simulink model "stereo_camera_q_dot"  (R2025b)
settings: Solver=FixedStepDiscrete  StartTime=0  StopTime=inf  FixedStep=Ts  RelTol=1e-3
InitFcn:
  | % 获取当前.slx模型所在文件夹
  | model_path = fileparts(which(gcs));
  | % 向上跳转、拼接目标函数所在文件夹（根据你的目录调整）
  | func_folder = fullfile(model_path,'..', 'config');
  | % 添加到搜索路径
  | addpath(func_folder);
  | % 执行初始化函数
  | init_single_camera_q_dot_tracking;
undefined symbols (not defined in the file or in its folder): camera_velocity_feedback_timeout_sec, controller_enable, cx, cy, data, data_SL_Info, depth_safe_max, depth_safe_min, depth_safety_gain, ekf_gate_threshold, enable_ekf_feedforward, enable_proportional, fx, fy, joint_acceleration_limit, joint_nominal_configuration, joint_position_max, joint_position_min, joint_soft_margin, joint_state_timeout_sec, joint_velocity_limit, k_ff, Kpx, Kpy, measurement_reset_timeout, nullspace_posture_gain, P0, Publish, Q_ekf, R_ekf, required_valid_frames, ros, ros2lib, singularity_sigma_stop, singularity_sigma_warn, Subscribe, target_timeout_sec, task_velocity_filter_tau, Ts, visual_damping_max, visual_damping_min, visual_min_depth, Z_hat
libraries: robotmaniplib x2
(part 1 of 2)
Description:
  | Fixed-focus monocular XY target tracking. Outputs camera-frame [vx vy 0 0 0 0]; robot kinematics remain external.
settings Model: DataDictionary=ros2lib.sldd  Creator=ASUS  LastModifiedBy=harry
settings DataIOCC: SignalLogging=off

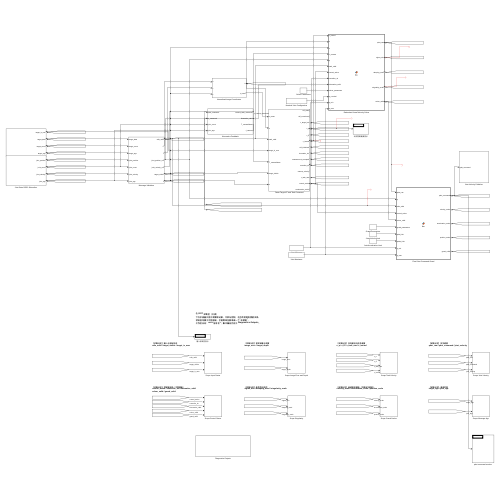
[thumbnail: Simulink's stored preview of the top-level diagram]
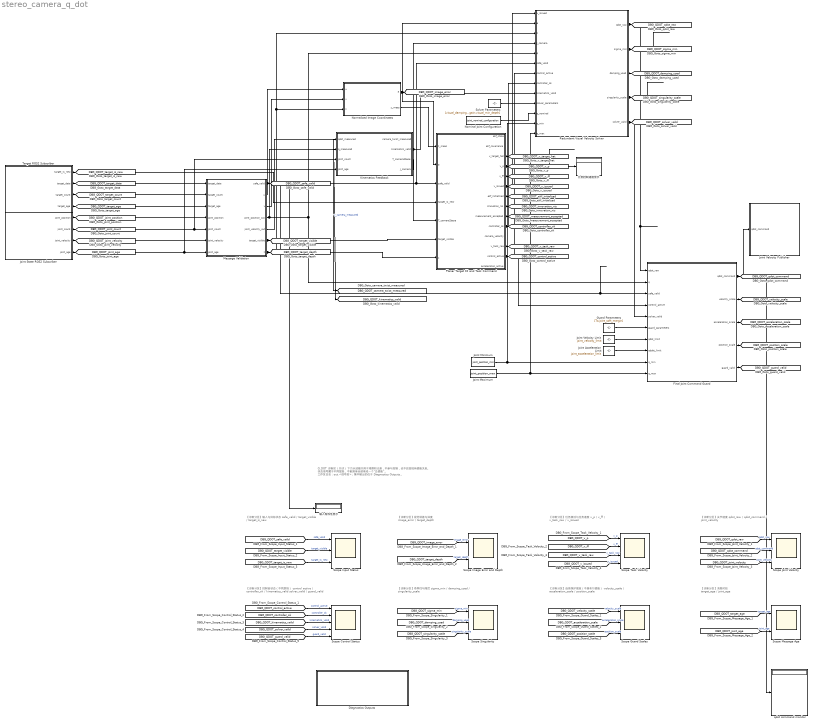
== system stereo_camera_q_dot ==
  note: Q_DOT 诊断区（只读）
      | 下方示波器只用于观察和记录，不参与控制，也不改变现有使能关系。
      | 状态信号属于不同层级，不能简单全部串成一个“总使能”。
      | 工作区日志：out.<信号名>；集中输出仍位于 Diagnostics Outputs。
  note: 【诊断分区】输入与目标状态
      | safe_valid / target_visible / target_is_new
  note: 【诊断分区】视觉误差与深度
      | image_error / target_depth
  note: 【诊断分区】任务激活与任务速度
      | v_p / v_ff / v_task_raw / v_issued
  note: 【诊断分区】关节速度
      | qdot_raw / qdot_command / joint_velocity
  note: 【诊断分区】控制链状态（不同层级）
      | control_active / controller_ok / kinematics_valid
      | solver_valid / guard_valid
  note: 【诊断分区】奇异性与阻尼
      | sigma_min / damping_used / singularity_scale
  note: 【诊断分区】连续保护缩放（不是布尔使能）
      | velocity_scale / acceleration_scale / position_scale
  note: 【诊断分区】消息时效
      | target_age / joint_age
  Diagnostics Outputs : Subsystem
  Final Joint Command Guard : MATLAB Function  TreatAsAtomicUnit=on
  Guard Parameters : Constant  Value=[Ts;joint_soft_margin]
  Joint Acceleration Limit : Constant  Value=joint_acceleration_limit
  Joint Maximum : Constant  Value=joint_position_max
  Joint Minimum : Constant  Value=joint_position_min
  Joint State ROS2 Subscriber : Subsystem
  Joint Velocity Limit : Constant  Value=joint_velocity_limit
  Joint Velocity Publisher : Subsystem
  Kinematics Feedback : Subsystem
  Message Validation : Subsystem
  Nominal Joint Configuration : Constant  Value=joint_nominal_configuration
  Normalized Image Coordinates : Subsystem
  Planar Target KF and Task Command : Subsystem
  Redundant Visual Velocity Solver : MATLAB Function  TreatAsAtomicUnit=on
  Scope Control Status : Scope  NumInputPorts=5
      settings: TimeSpan=10  ActiveDisplayString=5  Title=guard_valid  ActiveDisplayYMinimum=-0.037001953201183713  ActiveDisplayYMaximum=0.0101088347899616  DataLoggingVariableName=ScopeData4
  Scope Guard Scales : Scope  NumInputPorts=3
      settings: TimeSpan=10  ActiveDisplayString=3  Title=position_scale  ActiveDisplayYMinimum=-12.068513318672558  ActiveDisplayYMaximum=6.6876450330275015  DataLoggingVariableName=ScopeData6
  Scope Image Error and Depth : Scope  NumInputPorts=2
      settings: TimeSpan=10  Title=target_depth  ActiveDisplayYMinimum=-1  ActiveDisplayYMaximum=1
  Scope Input Status : Scope  NumInputPorts=3
      settings: TimeSpan=10  ActiveDisplayString=3  Title=target_is_new  ActiveDisplayYMinimum=-1.6084422447956979  ActiveDisplayYMaximum=1.406793571934575  DataLoggingVariableName=ScopeData7
  Scope Joint Velocity : Scope  NumInputPorts=3
      settings: TimeSpan=10  ActiveDisplayString=3  Title=joint_velocity  ActiveDisplayYMinimum=-1.0517167509781138  ActiveDisplayYMaximum=1.0307773782957734  DataLoggingVariableName=ScopeData2
  Scope Message Age : Scope  NumInputPorts=2
      settings: TimeSpan=10  Title=joint_age  ActiveDisplayYMinimum=-1  ActiveDisplayYMaximum=1
  Scope Singularity : Scope  NumInputPorts=3
      settings: TimeSpan=10  ActiveDisplayString=3  Title=singularity_scale  ActiveDisplayYMinimum=-3.3735923675324466  ActiveDisplayYMaximum=2.902388236211491  DataLoggingVariableName=ScopeData5
  Scope Task Velocity : Scope  NumInputPorts=4
      settings: TimeSpan=10  ActiveDisplayString=4  Title=v_issued  ActiveDisplayYMinimum=-1  ActiveDisplayYMaximum=1  DataLoggingVariableName=ScopeData3
  Solver Parameters : Constant  Value=[visual_damping_min;visual_damping_max;singularity_sigma_stop;singularity_sigma_warn;nullspace_posture_gain;depth_safe_min;depth_safe_max;depth_safety_gain;visual_min_depth]
  Target ROS2 Subscriber : Subsystem
  qdot command monitor : Display
  比例控制速度显示 : Display
  输入有效性显示 : Display
  tag scope: DBG_QDOT_acceleration_scale=global, DBG_QDOT_camera_twist_measured=global, DBG_QDOT_control_active=global, DBG_QDOT_controller_ok=global, DBG_QDOT_damping_used=global, DBG_QDOT_ekf_initialized=global, DBG_QDOT_guard_valid=global, DBG_QDOT_image_error=global, DBG_QDOT_innovation_nis=global, DBG_QDOT_joint_age=global, DBG_QDOT_joint_count=global, DBG_QDOT_joint_position=global, DBG_QDOT_joint_velocity=global, DBG_QDOT_kinematics_valid=global, DBG_QDOT_measurement_accepted=global, DBG_QDOT_position_scale=global, DBG_QDOT_qdot_command=global, DBG_QDOT_qdot_raw=global, DBG_QDOT_safe_valid=global, DBG_QDOT_sigma_min=global, DBG_QDOT_singularity_scale=global, DBG_QDOT_solver_valid=global, DBG_QDOT_target_age=global, DBG_QDOT_target_count=global, DBG_QDOT_target_data=global, DBG_QDOT_target_depth=global, DBG_QDOT_target_is_new=global, DBG_QDOT_target_visible=global, DBG_QDOT_v_ff=global, DBG_QDOT_v_issued=global, DBG_QDOT_v_p=global, DBG_QDOT_v_target_hat=global, DBG_QDOT_v_task_raw=global, DBG_QDOT_velocity_scale=global
  wires:
  Final Joint Command Guard/1(qdot_command) -> Joint Velocity Publisher/1(qdot_command), qdot command monitor/1, [DBG_QDOT_qdot_command]
  Message Validation/4(joint_position_out) -> Final Joint Command Guard/2(q), Redundant Visual Velocity Solver/5(q), Kinematics Feedback/2(q_measured)
  Kinematics Feedback/2(kinematics_valid) -> Redundant Visual Velocity Solver/9(kinematics_valid), [DBG_QDOT_kinematics_valid]
  Joint Velocity Limit/1 -> Final Joint Command Guard/7(qdot_limit)
  Message Validation/2(u) -> Normalized Image Coordinates/1(u)
  Target ROS2 Subscriber/3(target_count) -> Message Validation/2(target_count), [DBG_QDOT_target_count]
  Redundant Visual Velocity Solver/5(solver_valid) -> Final Joint Command Guard/5(solver_valid), [DBG_QDOT_solver_valid]
  Target ROS2 Subscriber/1(target_is_new) -> Planar Target KF and Task Command/4(target_is_new), [DBG_QDOT_target_is_new]
  Planar Target KF and Task Command/10(controller_ok) -> Redundant Visual Velocity Solver/8(controller_ok), [DBG_QDOT_controller_ok]
  Message Validation/5(joint_velocity_out) -> Kinematics Feedback/1(qdot_measured)
  Message Validation/7(z) -> Redundant Visual Velocity Solver/3(z), Normalized Image Coordinates/3(z), Planar Target KF and Task Command/7(z), [DBG_QDOT_target_depth]
  Joint Acceleration Limit/1 -> Final Joint Command Guard/8(qddot_limit)
  Joint State ROS2 Subscriber/4(joint_age) -> Kinematics Feedback/4(joint_age), Message Validation/7(joint_age), [DBG_QDOT_joint_age]
  Joint State ROS2 Subscriber/3(joint_velocity) -> Message Validation/6(joint_velocity), [DBG_QDOT_joint_velocity]
  Message Validation/6(target_visible) -> Planar Target KF and Task Command/6(target_visible), [DBG_QDOT_target_visible]
  Kinematics Feedback/4(J_camera) -> Redundant Visual Velocity Solver/4(J_camera)
  Redundant Visual Velocity Solver/1(qdot_raw) -> [DBG_QDOT_qdot_raw], Final Joint Command Guard/1(qdot_raw)
  Message Validation/1(safe_valid) -> Final Joint Command Guard/3(safe_valid), Redundant Visual Velocity Solver/6(safe_valid), Planar Target KF and Task Command/3(safe_valid), 输入有效性显示/1, [DBG_QDOT_safe_valid]
  Message Validation/3(v) -> Normalized Image Coordinates/2(v)
  Planar Target KF and Task Command/13(control_active) -> Redundant Visual Velocity Solver/7(control_active), Final Joint Command Guard/4(control_active), [DBG_QDOT_control_active]
  Joint State ROS2 Subscriber/1(joint_position) -> Message Validation/4(joint_position), [DBG_QDOT_joint_position]
  Guard Parameters/1 -> Final Joint Command Guard/6(guard_parameters)
  Joint State ROS2 Subscriber/2(joint_count) -> Kinematics Feedback/3(joint_count), Message Validation/5(joint_count), [DBG_QDOT_joint_count]
  Normalized Image Coordinates/1(e) -> Planar Target KF and Task Command/2(e), Redundant Visual Velocity Solver/2(e), [DBG_QDOT_image_error]
  Target ROS2 Subscriber/2(target_data) -> Message Validation/1(target_data), [DBG_QDOT_target_data]
  Normalized Image Coordinates/2(z_meas) -> Planar Target KF and Task Command/1(z_meas)
  Kinematics Feedback/3(T_camera2base) -> Planar Target KF and Task Command/5(T_camera2base)
  Solver Parameters/1 -> Redundant Visual Velocity Solver/10(solver_parameters)
  Nominal Joint Configuration/1 -> Redundant Visual Velocity Solver/11(q_nominal)
  Joint Minimum/1 -> Redundant Visual Velocity Solver/12(q_min), Final Joint Command Guard/9(q_min)
  Joint Maximum/1 -> Final Joint Command Guard/10(q_max), Redundant Visual Velocity Solver/13(q_max)
  Target ROS2 Subscriber/4(target_age) -> Message Validation/3(target_age), [DBG_QDOT_target_age]
  Planar Target KF and Task Command/4(v_p) -> 比例控制速度显示/1, [DBG_QDOT_v_p]
  Planar Target KF and Task Command/6(v_issued) -> Redundant Visual Velocity Solver/1(v_issued), [DBG_QDOT_v_issued]
  Redundant Visual Velocity Solver/2(sigma_min) -> [DBG_QDOT_sigma_min]
  Redundant Visual Velocity Solver/4(singularity_scale) -> [DBG_QDOT_singularity_scale]
  Kinematics Feedback/1(camera_twist_measured) -> [DBG_QDOT_camera_twist_measured]  "v_camera_measured"
  Planar Target KF and Task Command/3(v_target_hat) -> [DBG_QDOT_v_target_hat]
  Planar Target KF and Task Command/5(v_ff) -> [DBG_QDOT_v_ff]
  Planar Target KF and Task Command/7(ekf_initialized) -> [DBG_QDOT_ekf_initialized]
  Planar Target KF and Task Command/8(innovation_nis) -> [DBG_QDOT_innovation_nis]
  Planar Target KF and Task Command/9(measurement_accepted) -> [DBG_QDOT_measurement_accepted]
  Planar Target KF and Task Command/12(v_task_raw) -> [DBG_QDOT_v_task_raw]
  Redundant Visual Velocity Solver/3(damping_used) -> [DBG_QDOT_damping_used]
  Final Joint Command Guard/2(velocity_scale) -> [DBG_QDOT_velocity_scale]
  Final Joint Command Guard/3(acceleration_scale) -> [DBG_QDOT_acceleration_scale]
  Final Joint Command Guard/4(position_scale) -> [DBG_QDOT_position_scale]
  Final Joint Command Guard/5(guard_valid) -> [DBG_QDOT_guard_valid]
  [DBG_QDOT_safe_valid] -> Scope Input Status/1  "safe_valid"
  [DBG_QDOT_target_visible] -> Scope Input Status/2  "target_visible"
  [DBG_QDOT_target_is_new] -> Scope Input Status/3  "target_is_new"
  [DBG_QDOT_image_error] -> Scope Image Error and Depth/1  "image_error"
  [DBG_QDOT_target_depth] -> Scope Image Error and Depth/2  "target_depth"
  [DBG_QDOT_v_p] -> Scope Task Velocity/1  "v_p"
  [DBG_QDOT_v_ff] -> Scope Task Velocity/2  "v_ff"
  [DBG_QDOT_v_task_raw] -> Scope Task Velocity/3  "v_task_raw"
  [DBG_QDOT_v_issued] -> Scope Task Velocity/4  "v_issued"
  [DBG_QDOT_qdot_raw] -> Scope Joint Velocity/1  "qdot_raw"
  [DBG_QDOT_qdot_command] -> Scope Joint Velocity/2  "qdot_command"
  [DBG_QDOT_joint_velocity] -> Scope Joint Velocity/3  "joint_velocity"
  [DBG_QDOT_control_active] -> Scope Control Status/1  "control_active"
  [DBG_QDOT_controller_ok] -> Scope Control Status/2  "controller_ok"
  [DBG_QDOT_kinematics_valid] -> Scope Control Status/3  "kinematics_valid"
  [DBG_QDOT_solver_valid] -> Scope Control Status/4  "solver_valid"
  [DBG_QDOT_guard_valid] -> Scope Control Status/5  "guard_valid"
  [DBG_QDOT_sigma_min] -> Scope Singularity/1  "sigma_min"
  [DBG_QDOT_damping_used] -> Scope Singularity/2  "damping_used"
  [DBG_QDOT_singularity_scale] -> Scope Singularity/3  "singularity_scale"
  [DBG_QDOT_velocity_scale] -> Scope Guard Scales/1  "velocity_scale"
  [DBG_QDOT_acceleration_scale] -> Scope Guard Scales/2  "acceleration_scale"
  [DBG_QDOT_position_scale] -> Scope Guard Scales/3  "position_scale"
  [DBG_QDOT_target_age] -> Scope Message Age/1  "target_age"
  [DBG_QDOT_joint_age] -> Scope Message Age/2  "joint_age"

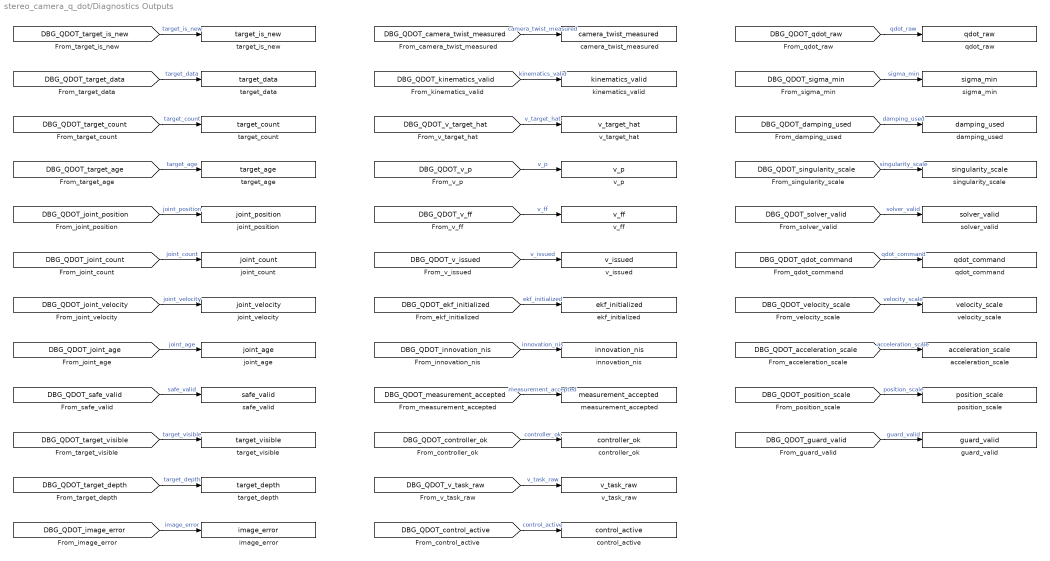
== system stereo_camera_q_dot/Diagnostics Outputs ==
  acceleration_scale : ToWorkspace  VariableName=acceleration_scale  SaveFormat=Timeseries  SampleTime=-1
  camera_twist_measured : ToWorkspace  VariableName=camera_twist_measured  SaveFormat=Timeseries  SampleTime=-1
  control_active : ToWorkspace  VariableName=control_active  SaveFormat=Timeseries  SampleTime=-1
  controller_ok : ToWorkspace  VariableName=controller_ok  SaveFormat=Timeseries  SampleTime=-1
  damping_used : ToWorkspace  VariableName=damping_used  SaveFormat=Timeseries  SampleTime=-1
  ekf_initialized : ToWorkspace  VariableName=ekf_initialized  SaveFormat=Timeseries  SampleTime=-1
  guard_valid : ToWorkspace  VariableName=guard_valid  SaveFormat=Timeseries  SampleTime=-1
  image_error : ToWorkspace  VariableName=image_error  SaveFormat=Timeseries  SampleTime=-1
  innovation_nis : ToWorkspace  VariableName=innovation_nis  SaveFormat=Timeseries  SampleTime=-1
  joint_age : ToWorkspace  VariableName=joint_age  SaveFormat=Timeseries  SampleTime=-1
  joint_count : ToWorkspace  VariableName=joint_count  SaveFormat=Timeseries  SampleTime=-1
  joint_position : ToWorkspace  VariableName=joint_position  SaveFormat=Timeseries  SampleTime=-1
  joint_velocity : ToWorkspace  VariableName=joint_velocity  SaveFormat=Timeseries  SampleTime=-1
  kinematics_valid : ToWorkspace  VariableName=kinematics_valid  SaveFormat=Timeseries  SampleTime=-1
  measurement_accepted : ToWorkspace  VariableName=measurement_accepted  SaveFormat=Timeseries  SampleTime=-1
  position_scale : ToWorkspace  VariableName=position_scale  SaveFormat=Timeseries  SampleTime=-1
  qdot_command : ToWorkspace  VariableName=qdot_command  SaveFormat=Timeseries  SampleTime=-1
  qdot_raw : ToWorkspace  VariableName=qdot_raw  SaveFormat=Timeseries  SampleTime=-1
  safe_valid : ToWorkspace  VariableName=safe_valid  SaveFormat=Timeseries  SampleTime=-1
  sigma_min : ToWorkspace  VariableName=sigma_min  SaveFormat=Timeseries  SampleTime=-1
  singularity_scale : ToWorkspace  VariableName=singularity_scale  SaveFormat=Timeseries  SampleTime=-1
  solver_valid : ToWorkspace  VariableName=solver_valid  SaveFormat=Timeseries  SampleTime=-1
  target_age : ToWorkspace  VariableName=target_age  SaveFormat=Timeseries  SampleTime=-1
  target_count : ToWorkspace  VariableName=target_count  SaveFormat=Timeseries  SampleTime=-1
  target_data : ToWorkspace  VariableName=target_data  SaveFormat=Timeseries  SampleTime=-1
  target_depth : ToWorkspace  VariableName=target_depth  SaveFormat=Timeseries  SampleTime=-1
  target_is_new : ToWorkspace  VariableName=target_is_new  SaveFormat=Timeseries  SampleTime=-1
  target_visible : ToWorkspace  VariableName=target_visible  SaveFormat=Timeseries  SampleTime=-1
  v_ff : ToWorkspace  VariableName=v_ff  SaveFormat=Timeseries  SampleTime=-1
  v_issued : ToWorkspace  VariableName=v_issued  SaveFormat=Timeseries  SampleTime=-1
  v_p : ToWorkspace  VariableName=v_p  SaveFormat=Timeseries  SampleTime=-1
  v_target_hat : ToWorkspace  VariableName=v_target_hat  SaveFormat=Timeseries  SampleTime=-1
  v_task_raw : ToWorkspace  VariableName=v_task_raw  SaveFormat=Timeseries  SampleTime=-1
  velocity_scale : ToWorkspace  VariableName=velocity_scale  SaveFormat=Timeseries  SampleTime=-1
  wires:
  [DBG_QDOT_target_is_new] -> target_is_new/1  "target_is_new"
  [DBG_QDOT_target_data] -> target_data/1  "target_data"
  [DBG_QDOT_target_count] -> target_count/1  "target_count"
  [DBG_QDOT_target_age] -> target_age/1  "target_age"
  [DBG_QDOT_joint_position] -> joint_position/1  "joint_position"
  [DBG_QDOT_joint_count] -> joint_count/1  "joint_count"
  [DBG_QDOT_joint_velocity] -> joint_velocity/1  "joint_velocity"
  [DBG_QDOT_joint_age] -> joint_age/1  "joint_age"
  [DBG_QDOT_safe_valid] -> safe_valid/1  "safe_valid"
  [DBG_QDOT_target_visible] -> target_visible/1  "target_visible"
  [DBG_QDOT_target_depth] -> target_depth/1  "target_depth"
  [DBG_QDOT_image_error] -> image_error/1  "image_error"
  [DBG_QDOT_camera_twist_measured] -> camera_twist_measured/1  "camera_twist_measured"
  [DBG_QDOT_kinematics_valid] -> kinematics_valid/1  "kinematics_valid"
  [DBG_QDOT_v_target_hat] -> v_target_hat/1  "v_target_hat"
  [DBG_QDOT_v_p] -> v_p/1  "v_p"
  [DBG_QDOT_v_ff] -> v_ff/1  "v_ff"
  [DBG_QDOT_v_issued] -> v_issued/1  "v_issued"
  [DBG_QDOT_ekf_initialized] -> ekf_initialized/1  "ekf_initialized"
  [DBG_QDOT_innovation_nis] -> innovation_nis/1  "innovation_nis"
  [DBG_QDOT_measurement_accepted] -> measurement_accepted/1  "measurement_accepted"
  [DBG_QDOT_controller_ok] -> controller_ok/1  "controller_ok"
  [DBG_QDOT_v_task_raw] -> v_task_raw/1  "v_task_raw"
  [DBG_QDOT_control_active] -> control_active/1  "control_active"
  [DBG_QDOT_qdot_raw] -> qdot_raw/1  "qdot_raw"
  [DBG_QDOT_sigma_min] -> sigma_min/1  "sigma_min"
  [DBG_QDOT_damping_used] -> damping_used/1  "damping_used"
  [DBG_QDOT_singularity_scale] -> singularity_scale/1  "singularity_scale"
  [DBG_QDOT_solver_valid] -> solver_valid/1  "solver_valid"
  [DBG_QDOT_qdot_command] -> qdot_command/1  "qdot_command"
  [DBG_QDOT_velocity_scale] -> velocity_scale/1  "velocity_scale"
  [DBG_QDOT_acceleration_scale] -> acceleration_scale/1  "acceleration_scale"
  [DBG_QDOT_position_scale] -> position_scale/1  "position_scale"
  [DBG_QDOT_guard_valid] -> guard_valid/1  "guard_valid"

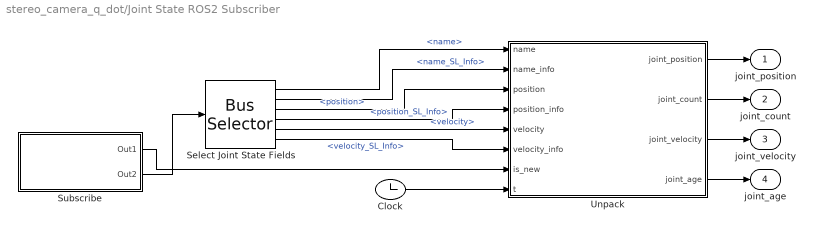
== system stereo_camera_q_dot/Joint State ROS2 Subscriber ==
  Clock : Clock
  Select Joint State Fields : BusSelector  OutputSignals=name,name_SL_Info,position,position_SL_Info,velocity,velocity_SL_Info
  Subscribe : Subsystem  AncestorBlock=ros2lib/Subscribe  LoadFcn=ros.slros2.internal.block.SubscribeBlockMask.messageLoadFcn(gcb);  InitFcn=ros.slros.internal.block.errorIfBlocksConflict(bdroot(gcb));  mask(ROS2 Subscribe){topicSource=Select from ROS network, topic=/franka/joint_states, messageType=sensor_msgs/JointState, sampleTime=Ts, QOSHistory=Keep last, QOSDepth=1, QOSReliability=Best effort, QOSDurability=Volatile, QOSDeadline=Inf, QOSLifespan=Inf, QOSLiveliness=Automatic, QOSLeaseDuration=Inf, QOSAvoidROSNamespaceConventions=off}
      mask prompts: topicSource "ros:slros:blockmask:TopicSourcePrompt"; topic "ros:slros:blockmask:TopicPrompt"; messageType "ros:slros:blockmask:MessageTypePrompt"; sampleTime "ros:slros:blockmask:SampleTimePrompt"; QOSHistory "ros:slros2:blockmask:QOSHistoryPrompt"; QOSDepth "ros:slros2:blockmask:QOSDepthPrompt"; QOSReliability "ros:slros2:blockmask:QOSReliabilityPrompt"; QOSDurability "ros:slros2:blockmask:QOSDurabilityPrompt"; QOSDeadline "ros:slros2:blockmask:QOSDeadlinePrompt"; QOSLifespan "ros:slros2:blockmask:QOSLifespanPrompt"; QOSLiveliness "ros:slros2:blockmask:QOSLivelinessPrompt"; QOSLeaseDuration "ros:slros2:blockmask:QOSLeaseDurationPrompt"; QOSAvoidROSNamespaceConventions "ros:slros2:blockmask:QOSAvoidROSNamespaceConventionsPrompt"
      mask help: ros:slros:blockmask:SubscriberDescription
      mask init:
      | ros.slros2.internal.block.SubscribeBlockMask.dispatch('maskInitialize', gcb);
      settings: ModelCloseFcn=ros.slros2.internal.bus.Util.clearSLBusesInGlobalScope(gcb);
      mask Help: eval('ros.slros.internal.helpview(''ros2SubscribeBlock'')');
      mask TypeOptions topicSource: ros:slros2:blockmask:TopicSourceFromNetwork | ros:slros2:blockmask:TopicSourceSpecifyOwn
      mask Callback topicSource: ros.slros2.internal.block.SubscribeBlockMask.dispatch('topicSourceSelect', gcb);
      mask Callback topic: ros.slros2.internal.block.SubscribeBlockMask.dispatch('topicEdit', gcb);
      mask Callback messageType: ros.slros2.internal.block.SubscribeBlockMask.dispatch('messageTypeEdit', gcb);
      mask TypeOptions sampleTime: Constant/SampleTime
      mask TypeOptions QOSHistory: SourceBlock/QOSHistory
      mask Callback QOSHistory: ros.slros2.internal.block.QOSSettingsMask.qosHistorySelect(gcb);
      mask TypeOptions QOSDepth: SourceBlock/QOSDepth
      mask TypeOptions QOSReliability: SourceBlock/QOSReliability
      mask TypeOptions QOSDurability: SourceBlock/QOSDurability
      mask TypeOptions QOSDeadline: SourceBlock/QOSDeadline
      mask TypeOptions QOSLifespan: SourceBlock/QOSLifespan
      mask TypeOptions QOSLiveliness: SourceBlock/QOSLiveliness
      mask TypeOptions QOSLeaseDuration: SourceBlock/QOSLeaseDuration
      mask TypeOptions QOSAvoidROSNamespaceConventions: SourceBlock/QOSAvoidROSNamespaceConventions
      mask DialogControl id_netAddrLink Prompt: ros:slros2:blockmask:ConfigNetworkAddrLinkText
      mask DialogControl id_netAddrLink Callback: ros.slros2.internal.block.SubscribeBlockMask.dispatch('configureNetworkAddrDlg', gcb);
      mask DialogControl Container13 Prompt: ros:slros2:blockmask:PubSubMainTab
      mask DialogControl topicSource Prompt: Topic source:
      mask DialogControl topic Prompt: Topic:
      mask DialogControl id_topicSelectBtn Prompt: ros:slros:blockmask:SelectPrompt
      mask DialogControl id_topicSelectBtn Callback: ros.slros2.internal.block.SubscribeBlockMask.dispatch('topicSelect', gcb, 'ros.slros2.internal.dlg.TopicSelector');
      mask DialogControl messageType Prompt: Message type:
      mask DialogControl id_msgTypeSelectBtn Prompt: ros:slros:blockmask:SelectPrompt
      mask DialogControl id_msgTypeSelectBtn Callback: ros.slros2.internal.block.SubscribeBlockMask.dispatch('messageTypeSelect', gcb, 'ros.slros2.internal.dlg.MessageTypeSelector');
      mask DialogControl sampleTime Prompt: Sample time:
      mask DialogControl id_cgContainer Prompt: ros:slros2:blockmask:PubSubQOSTab
      mask DialogControl QOSHistory Prompt: History:
      mask DialogControl QOSDepth Prompt: Depth:
      mask DialogControl QOSReliability Prompt: Reliability:
      mask DialogControl QOSDurability Prompt: Durability:
      mask DialogControl QOSDeadline Prompt: Deadline:
      mask DialogControl QOSLifespan Prompt: Lifespan:
      mask DialogControl QOSLiveliness Prompt: Liveliness:
      mask DialogControl QOSLeaseDuration Prompt: Lease Duration:
      mask DialogControl QOSAvoidROSNamespaceConventions Prompt: Avoid ROS Namespace Conventions
      mask Display:
      | color('black');
      | text(0.83, 0.15, '/franka/joint_states', 'horizontalAlignment', 'right');
      | port_label('output', 1, 'IsNew');
      | port_label('output', 2, 'Msg');
  Unpack : MATLAB Function  TreatAsAtomicUnit=on
  joint_position : Outport
  joint_count : Outport  Port=2
  joint_velocity : Outport  Port=3
  joint_age : Outport  Port=4
  wires:
  Unpack/1(joint_position) -> joint_position/1
  Unpack/2(joint_count) -> joint_count/1
  Unpack/3(joint_velocity) -> joint_velocity/1
  Unpack/4(joint_age) -> joint_age/1
  Subscribe/2(Out2) -> Select Joint State Fields/1
  Select Joint State Fields/1 -> Unpack/1(name)  "<name>"
  Select Joint State Fields/2 -> Unpack/2(name_info)  "<name_SL_Info>"
  Select Joint State Fields/3 -> Unpack/3(position)  "<position>"
  Select Joint State Fields/4 -> Unpack/4(position_info)  "<position_SL_Info>"
  Select Joint State Fields/5 -> Unpack/5(velocity)  "<velocity>"
  Select Joint State Fields/6 -> Unpack/6(velocity_info)  "<velocity_SL_Info>"
  Subscribe/1(Out1) -> Unpack/7(is_new)
  Clock/1 -> Unpack/8(t)

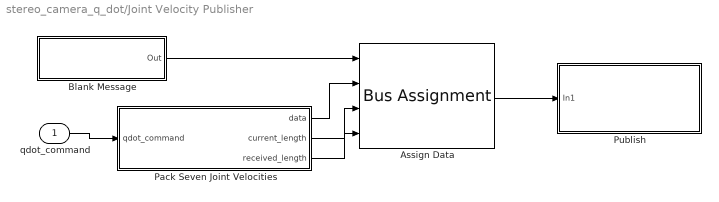
== system stereo_camera_q_dot/Joint Velocity Publisher ==
  qdot_command : Inport
  Assign Data : BusAssignment  AssignedSignals=data,data_SL_Info.CurrentLength,data_SL_Info.ReceivedLength
  Blank Message : Subsystem  AncestorBlock=ros2lib/Blank Message  LoadFcn=ros.slros2.internal.block.MessageBlockMask.messageLoadFcn(gcb);  InitFcn=ros.slros.internal.block.errorIfBlocksConflict(bdroot(gcb));  mask(ROS2 Blank Message){messageClass=Message, entityType=std_msgs/Float64MultiArray, messageType=std_msgs/Float64MultiArray, SampleTime=Ts}
      mask prompts: messageClass "ros:slros:blockmask:MessageClassPrompt"; entityType "ros:slros:blockmask:TypePrompt"; messageType "ros:slros:blockmask:FullTypePrompt"; SampleTime "Simulink:blkprm_prompts:AllSrcBlksSampleTime"
      mask help: ros:slros2:blockmask:BlankMsgDescription
      mask init:
      | ros.slros2.internal.block.MessageBlockMask.dispatch('maskInitialize', gcb);
      settings: ModelCloseFcn=ros.slros2.internal.bus.Util.clearSLBusesInGlobalScope(gcb);
      mask Help: eval('ros.slros.internal.helpview(''ros2BlankMsgBlock'')');
      mask TypeOptions messageClass: ros:slros:blockmask:MessageType_Msg | ros:slros:blockmask:MessageType_SrvReq | ros:slros:blockmask:MessageType_SrvResp | ros:slros:blockmask:MessageType_ActFb | ros:slros:blockmask:MessageType_ActGoal | ros:slros:blockmask:MessageType_ActRes
      mask Callback messageClass: ros.slros2.internal.block.MessageBlockMask.dispatch('messageClassChange', gcb);
      mask Callback entityType: ros.slros2.internal.block.MessageBlockMask.dispatch('entityTypeEdit', gcb);
      mask TypeOptions SampleTime: Constant/SampleTime
      mask DialogControl messageClass Prompt: Class:
      mask DialogControl entityType Prompt: Type:
      mask DialogControl id_msgTypeSelectBtn Prompt: ros:slros:blockmask:SelectPrompt
      mask DialogControl id_msgTypeSelectBtn Callback: ros.slros2.internal.block.MessageBlockMask.dispatch('selectButtonPressed', gcb);
      mask DialogControl messageType Prompt: Fully resolved type:
      mask DialogControl SampleTime Prompt: 采样时间:
      mask Display:
      | color('black');
      | text(0.96, 0.15, 'std_msgs/Float64MultiArray', 'horizontalAlignment', 'right');
  Pack Seven Joint Velocities : MATLAB Function  TreatAsAtomicUnit=on
  Publish : Subsystem  AncestorBlock=ros2lib/Publish  LoadFcn=ros.slros2.internal.block.PublishBlockMask.messageLoadFcn(gcb);  InitFcn=ros.slros.internal.block.errorIfBlocksConflict(bdroot(gcb));  mask(ROS2 Publish){topicSource=Select from ROS network, topic=/joint_velocity_example_controller/commands, messageType=std_msgs/Float64MultiArray, QOSHistory=Keep last, QOSDepth=1, QOSReliability=Reliable, QOSDurability=Volatile, QOSDeadline=Inf, QOSLifespan=Inf, QOSLiveliness=Automatic, QOSLeaseDuration=Inf, QOSAvoidROSNamespaceConventions=off}
      mask prompts: topicSource "ros:slros:blockmask:TopicSourcePrompt"; topic "ros:slros:blockmask:TopicPrompt"; messageType "ros:slros:blockmask:MessageTypePrompt"; QOSHistory "ros:slros2:blockmask:QOSHistoryPrompt"; QOSDepth "ros:slros2:blockmask:QOSDepthPrompt"; QOSReliability "ros:slros2:blockmask:QOSReliabilityPrompt"; QOSDurability "ros:slros2:blockmask:QOSDurabilityPrompt"; QOSDeadline "ros:slros2:blockmask:QOSDeadlinePrompt"; QOSLifespan "ros:slros2:blockmask:QOSLifespanPrompt"; QOSLiveliness "ros:slros2:blockmask:QOSLivelinessPrompt"; QOSLeaseDuration "ros:slros2:blockmask:QOSLeaseDurationPrompt"; QOSAvoidROSNamespaceConventions "ros:slros2:blockmask:QOSAvoidROSNamespaceConventionsPrompt"
      mask help: ros:slros:blockmask:PublisherDescription
      mask init:
      | ros.slros2.internal.block.PublishBlockMask.dispatch('maskInitialize', gcb);
      settings: ModelCloseFcn=ros.slros2.internal.bus.Util.clearSLBusesInGlobalScope(gcb);
      mask Help: eval('ros.slros.internal.helpview(''ros2PublishBlock'')');
      mask TypeOptions topicSource: ros:slros2:blockmask:TopicSourceFromNetwork | ros:slros2:blockmask:TopicSourceSpecifyOwn
      mask Callback topicSource: ros.slros2.internal.block.PublishBlockMask.dispatch('topicSourceSelect', gcb);
      mask Callback topic: ros.slros2.internal.block.PublishBlockMask.dispatch('topicEdit', gcb);
      mask Callback messageType: ros.slros2.internal.block.PublishBlockMask.dispatch('messageTypeEdit', gcb);
      mask TypeOptions QOSHistory: SinkBlock/QOSHistory
      mask Callback QOSHistory: ros.slros2.internal.block.QOSSettingsMask.qosHistorySelect(gcb);
      mask TypeOptions QOSDepth: SinkBlock/QOSDepth
      mask TypeOptions QOSReliability: SinkBlock/QOSReliability
      mask TypeOptions QOSDurability: SinkBlock/QOSDurability
      mask TypeOptions QOSDeadline: SinkBlock/QOSDeadline
      mask TypeOptions QOSLifespan: SinkBlock/QOSLifespan
      mask TypeOptions QOSLiveliness: SinkBlock/QOSLiveliness
      mask TypeOptions QOSLeaseDuration: SinkBlock/QOSLeaseDuration
      mask TypeOptions QOSAvoidROSNamespaceConventions: SinkBlock/QOSAvoidROSNamespaceConventions
      mask DialogControl id_netAddrLink Prompt: ros:slros2:blockmask:ConfigNetworkAddrLinkText
      mask DialogControl id_netAddrLink Callback: ros.slros2.internal.block.PublishBlockMask.dispatch('configureNetworkAddrDlg', gcb);
      mask DialogControl Container13 Prompt: ros:slros2:blockmask:PubSubMainTab
      mask DialogControl topicSource Prompt: Topic source:
      mask DialogControl topic Prompt: Topic:
      mask DialogControl id_topicSelectBtn Prompt: ros:slros:blockmask:SelectPrompt
      mask DialogControl id_topicSelectBtn Callback: ros.slros2.internal.block.PublishBlockMask.dispatch('topicSelect', gcb, 'ros.slros2.internal.dlg.TopicSelector');
      mask DialogControl messageType Prompt: Message type:
      mask DialogControl id_msgTypeSelectBtn Prompt: ros:slros:blockmask:SelectPrompt
      mask DialogControl id_msgTypeSelectBtn Callback: ros.slros2.internal.block.PublishBlockMask.dispatch('messageTypeSelect', gcb, 'ros.slros2.internal.dlg.MessageTypeSelector');
      mask DialogControl id_cgContainer Prompt: ros:slros2:blockmask:PubSubQOSTab
      mask DialogControl QOSHistory Prompt: History:
      mask DialogControl QOSDepth Prompt: Depth:
      mask DialogControl QOSReliability Prompt: Reliability:
      mask DialogControl QOSDurability Prompt: Durability:
      mask DialogControl QOSDeadline Prompt: Deadline:
      mask DialogControl QOSLifespan Prompt: Lifespan:
      mask DialogControl QOSLiveliness Prompt: Liveliness:
      mask DialogControl QOSLeaseDuration Prompt: Lease Duration:
      mask DialogControl QOSAvoidROSNamespaceConventions Prompt: Avoid ROS Namespace Conventions
      mask Display:
      | color('black');
      | text(0.83, 0.15, '/joint_velocity_example_controller/commands', 'horizontalAlignment', 'right');
  wires:
  ? -> ?
  qdot_command/1 -> Pack Seven Joint Velocities/1(qdot_command)
  Blank Message/1(Out) -> Assign Data/1
  Pack Seven Joint Velocities/1(data) -> Assign Data/2
  Pack Seven Joint Velocities/2(current_length) -> Assign Data/3
  Pack Seven Joint Velocities/3(received_length) -> Assign Data/4
  Assign Data/1 -> Publish/1(In1)

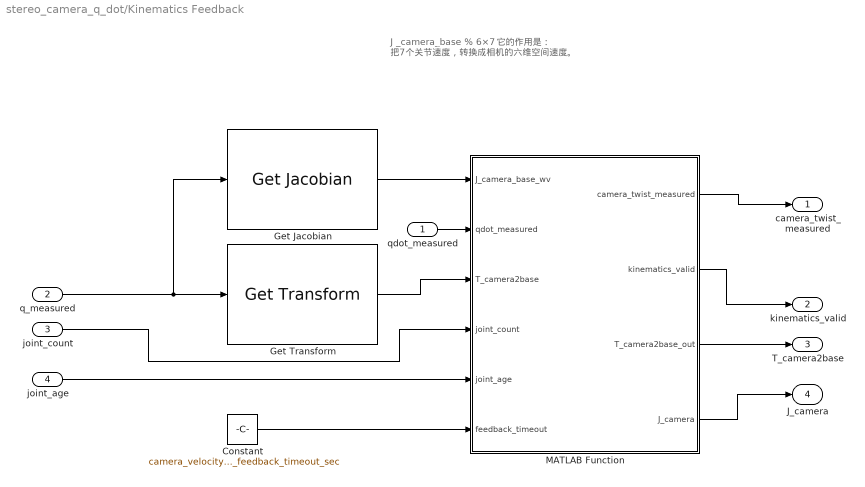
== system stereo_camera_q_dot/Kinematics Feedback ==
  note: J _camera_base % 6×7
      | 它的作用是：
      | 把7个关节速度，转换成相机的六维空间速度。
  qdot_measured : Inport
  q_measured : Inport  Port=2
  joint_count : Inport  Port=3
  joint_age : Inport  Port=4
  Constant : Constant  Value=camera_velocity_feedback_timeout_sec
  Get Jacobian : robotmaniplib/Get Jacobian  RigidBodyTree=fr3_camera_robot  EndEffector=camera_link  SimulateUsing=Interpreted execution
  Get Transform : robotmaniplib/Get Transform  RigidBodyTree=fr3_camera_robot  SourceBody=camera_link  TargetBody=base  SimulateUsing=Interpreted execution
  MATLAB Function : MATLAB Function  TreatAsAtomicUnit=on
  camera_twist_measured : Outport
  kinematics_valid : Outport  Port=2
  T_camera2base : Outport  Port=3
  J_camera : Outport  Port=4
  wires:
  q_measured/1 -> Get Jacobian/1, Get Transform/1
  qdot_measured/1 -> MATLAB Function/2(qdot_measured)
  Get Jacobian/1 -> MATLAB Function/1(J_camera_base_wv)
  Get Transform/1 -> MATLAB Function/3(T_camera2base)
  joint_count/1 -> MATLAB Function/4(joint_count)
  joint_age/1 -> MATLAB Function/5(joint_age)
  Constant/1 -> MATLAB Function/6(feedback_timeout)
  MATLAB Function/1(camera_twist_measured) -> camera_twist_measured/1
  MATLAB Function/2(kinematics_valid) -> kinematics_valid/1
  MATLAB Function/3(T_camera2base_out) -> T_camera2base/1
  MATLAB Function/4(J_camera) -> J_camera/1

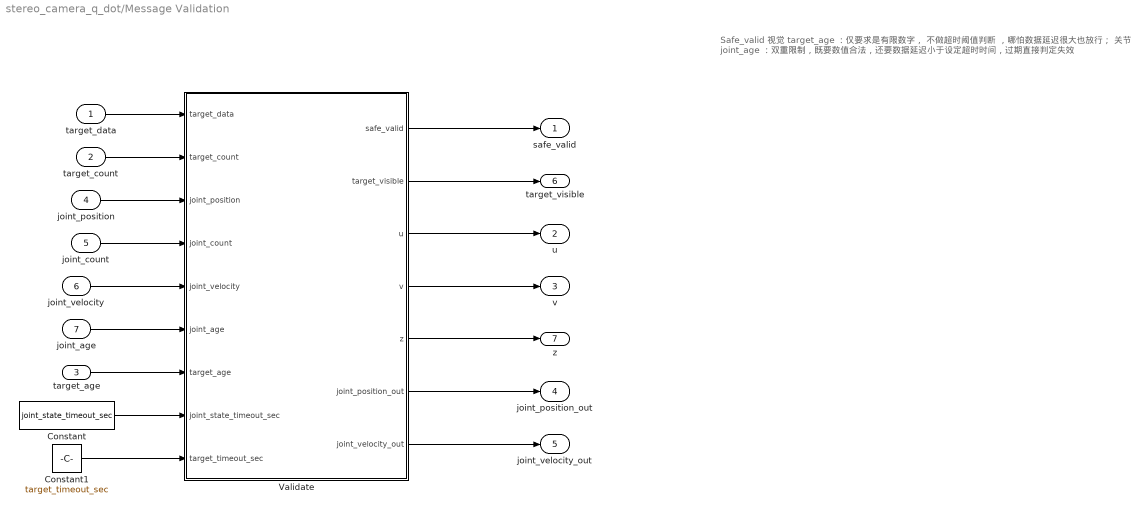
== system stereo_camera_q_dot/Message Validation ==
  note: Safe_valid
      | 视觉 target_age ：仅要求是有限数字， 不做超时阈值判断 ，哪怕数据延迟很大也放行；
      | 关节 joint_age ：双重限制，既要数值合法，还要数据延迟小于设定超时时间，过期直接判定失效
  target_data : Inport
  target_count : Inport  Port=2
  target_age : Inport  Port=3
  joint_position : Inport  Port=4
  joint_count : Inport  Port=5
  joint_velocity : Inport  Port=6
  joint_age : Inport  Port=7
  Constant : Constant  Value=joint_state_timeout_sec
  Constant1 : Constant  Value=target_timeout_sec
  Validate : MATLAB Function  TreatAsAtomicUnit=on
  safe_valid : Outport
  u : Outport  Port=2
  v : Outport  Port=3
  joint_position_out : Outport  Port=4
  joint_velocity_out : Outport  Port=5
  target_visible : Outport  Port=6
  z : Outport  Port=7
  wires:
  Validate/1(safe_valid) -> safe_valid/1
  Validate/3(u) -> u/1
  Validate/4(v) -> v/1
  Validate/6(joint_position_out) -> joint_position_out/1
  Validate/7(joint_velocity_out) -> joint_velocity_out/1
  target_data/1 -> Validate/1(target_data)
  target_count/1 -> Validate/2(target_count)
  Validate/2(target_visible) -> target_visible/1
  joint_position/1 -> Validate/3(joint_position)
  joint_count/1 -> Validate/4(joint_count)
  joint_velocity/1 -> Validate/5(joint_velocity)
  joint_age/1 -> Validate/6(joint_age)
  Constant/1 -> Validate/8(joint_state_timeout_sec)
  Validate/5(z) -> z/1
  target_age/1 -> Validate/7(target_age)
  Constant1/1 -> Validate/9(target_timeout_sec)

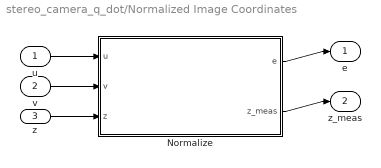
== system stereo_camera_q_dot/Normalized Image Coordinates ==
  u : Inport
  v : Inport  Port=2
  z : Inport  Port=3
  Normalize : MATLAB Function  TreatAsAtomicUnit=on
  e : Outport
  z_meas : Outport  Port=2
  wires:
  u/1 -> Normalize/1(u)
  v/1 -> Normalize/2(v)
  Normalize/1(e) -> e/1
  Normalize/2(z_meas) -> z_meas/1
  z/1 -> Normalize/3(z)

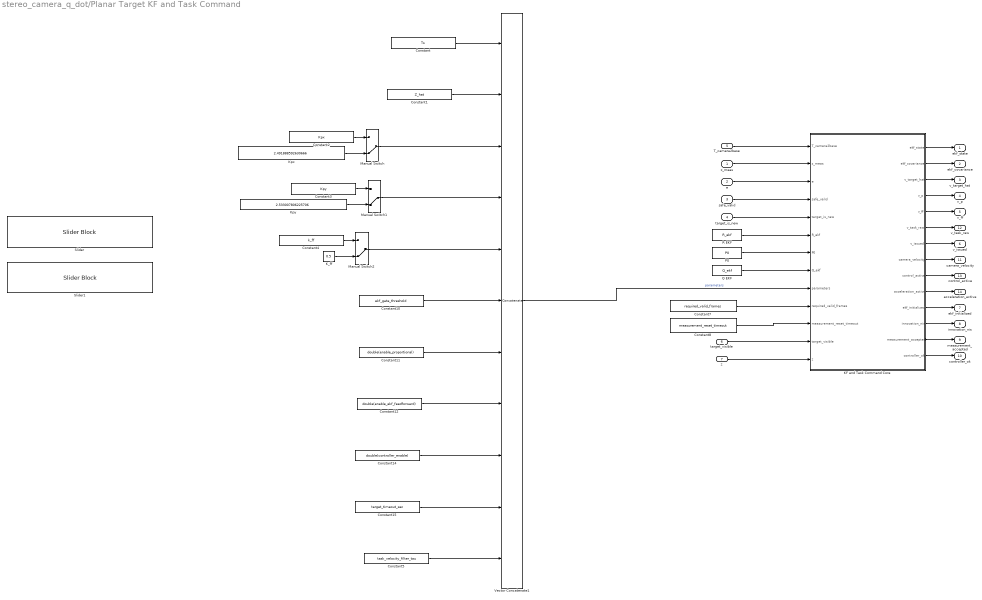
== system stereo_camera_q_dot/Planar Target KF and Task Command ==
  z_meas : Inport
  e : Inport  Port=2
  safe_valid : Inport  Port=3
  target_is_new : Inport  Port=4
  T_camera2base : Inport  Port=5
  target_visible : Inport  Port=6
  z : Inport  Port=7
  Constant : Constant  Value=Ts
  Constant1 : Constant  Value=Z_hat
  Constant10 : Constant  Value=ekf_gate_threshold
  Constant11 : Constant  Value=double(enable_proportional)
  Constant12 : Constant  Value=double(enable_ekf_feedforward)
  Constant14 : Constant  Value=double(controller_enable)
  Constant15 : Constant  Value=target_timeout_sec
  Constant2 : Constant  Value=Kpx
  Constant3 : Constant  Value=Kpy
  Constant4 : Constant  Value=k_ff
  Constant5 : Constant  Value=task_velocity_filter_tau
  Constant7 : Constant  Value=required_valid_frames
  Constant8 : Constant  Value=measurement_reset_timeout
  KF and Task Command Core : MATLAB Function  TreatAsAtomicUnit=on
  K_ff : Constant  Value=0.5
  Kpx : Constant  Value=2.491888592630666
  Kpy : Constant  Value=2.533007806225706
  Manual Switch : ManualSwitch  CurrentSetting=0
  Manual Switch1 : ManualSwitch  CurrentSetting=0
  Manual Switch2 : ManualSwitch  CurrentSetting=0
  P0 : Constant  Value=P0
  Q EKF : Constant  Value=Q_ekf
  R EKF : Constant  Value=R_ekf
  Slider : SliderBlock  ScaleMax=10
  Slider1 : SliderBlock  ScaleMax=10
  Vector Concatenate1 : Concatenate  NumInputs=11
  ekf_state : Outport
  ekf_covariance : Outport  Port=2
  v_target_hat : Outport  Port=3
  v_p : Outport  Port=4
  v_ff : Outport  Port=5
  v_issued : Outport  Port=6
  ekf_initialized : Outport  Port=7
  innovation_nis : Outport  Port=8
  measurement_accepted : Outport  Port=9
  controller_ok : Outport  Port=10
  camera_velocity : Outport  Port=11
  v_task_raw : Outport  Port=12
  control_active : Outport  Port=13
  acceleration_active : Outport  Port=14
  wires:
  KF and Task Command Core/1(ekf_state) -> ekf_state/1
  KF and Task Command Core/2(ekf_covariance) -> ekf_covariance/1
  KF and Task Command Core/3(v_target_hat) -> v_target_hat/1
  KF and Task Command Core/4(v_p) -> v_p/1
  KF and Task Command Core/5(v_ff) -> v_ff/1
  KF and Task Command Core/7(v_issued) -> v_issued/1
  KF and Task Command Core/8(camera_velocity) -> camera_velocity/1
  KF and Task Command Core/11(ekf_initialized) -> ekf_initialized/1
  KF and Task Command Core/12(innovation_nis) -> innovation_nis/1
  KF and Task Command Core/13(measurement_accepted) -> measurement_accepted/1
  KF and Task Command Core/14(controller_ok) -> controller_ok/1
  z_meas/1 -> KF and Task Command Core/2(z_meas)
  e/1 -> KF and Task Command Core/3(e)
  safe_valid/1 -> KF and Task Command Core/4(safe_valid)
  target_is_new/1 -> KF and Task Command Core/5(target_is_new)
  Vector Concatenate1/1 -> KF and Task Command Core/9(parameters)  "parameters"
  P0/1 -> KF and Task Command Core/7(P0)
  Q EKF/1 -> KF and Task Command Core/8(Q_ekf)
  R EKF/1 -> KF and Task Command Core/6(R_ekf)
  Constant/1 -> Vector Concatenate1/1
  Constant1/1 -> Vector Concatenate1/2
  Constant10/1 -> Vector Concatenate1/6
  Constant11/1 -> Vector Concatenate1/7
  Constant12/1 -> Vector Concatenate1/8
  Constant14/1 -> Vector Concatenate1/9
  Constant15/1 -> Vector Concatenate1/10
  T_camera2base/1 -> KF and Task Command Core/1(T_camera2base)
  Constant2/1 -> Manual Switch/1
  Manual Switch/1 -> Vector Concatenate1/3
  Kpx/1 -> Manual Switch/2
  Kpy/1 -> Manual Switch1/2
  Constant3/1 -> Manual Switch1/1
  Manual Switch1/1 -> Vector Concatenate1/4
  Constant4/1 -> Manual Switch2/1
  Manual Switch2/1 -> Vector Concatenate1/5
  K_ff/1 -> Manual Switch2/2
  KF and Task Command Core/6(v_task_raw) -> v_task_raw/1
  KF and Task Command Core/10(acceleration_active) -> acceleration_active/1
  KF and Task Command Core/9(control_active) -> control_active/1
  ? -> ?
  ? -> ?
  Constant7/1 -> KF and Task Command Core/10(required_valid_frames)
  Constant8/1 -> KF and Task Command Core/11(measurement_reset_timeout)
  target_visible/1 -> KF and Task Command Core/12(target_visible)
  z/1 -> KF and Task Command Core/13(z)
  Constant5/1 -> Vector Concatenate1/11

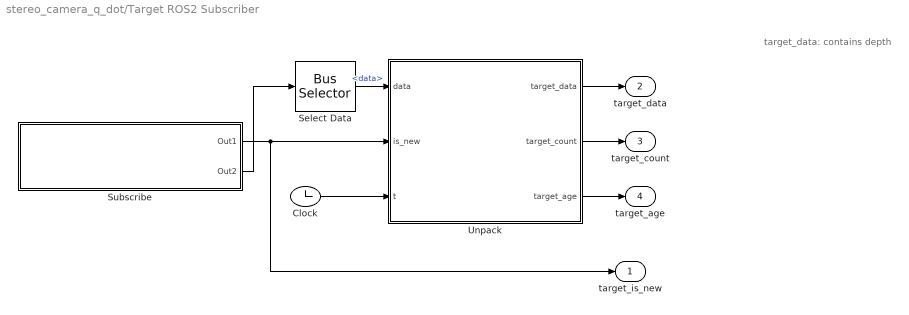
== system stereo_camera_q_dot/Target ROS2 Subscriber ==
  note: target_data: contains depth
  Clock : Clock
  Select Data : BusSelector  OutputSignals=data
  Subscribe : Subsystem  AncestorBlock=ros2lib/Subscribe  LoadFcn=ros.slros2.internal.block.SubscribeBlockMask.messageLoadFcn(gcb);  InitFcn=ros.slros.internal.block.errorIfBlocksConflict(bdroot(gcb));  mask(ROS2 Subscribe){topicSource=Select from ROS network, topic=/apriltag_detector/target_position, messageType=std_msgs/Float64MultiArray, sampleTime=Ts, QOSHistory=Keep last, QOSDepth=1, QOSReliability=Best effort, QOSDurability=Volatile, QOSDeadline=Inf, QOSLifespan=Inf, QOSLiveliness=Automatic, QOSLeaseDuration=Inf, QOSAvoidROSNamespaceConventions=off}
      mask prompts: topicSource "ros:slros:blockmask:TopicSourcePrompt"; topic "ros:slros:blockmask:TopicPrompt"; messageType "ros:slros:blockmask:MessageTypePrompt"; sampleTime "ros:slros:blockmask:SampleTimePrompt"; QOSHistory "ros:slros2:blockmask:QOSHistoryPrompt"; QOSDepth "ros:slros2:blockmask:QOSDepthPrompt"; QOSReliability "ros:slros2:blockmask:QOSReliabilityPrompt"; QOSDurability "ros:slros2:blockmask:QOSDurabilityPrompt"; QOSDeadline "ros:slros2:blockmask:QOSDeadlinePrompt"; QOSLifespan "ros:slros2:blockmask:QOSLifespanPrompt"; QOSLiveliness "ros:slros2:blockmask:QOSLivelinessPrompt"; QOSLeaseDuration "ros:slros2:blockmask:QOSLeaseDurationPrompt"; QOSAvoidROSNamespaceConventions "ros:slros2:blockmask:QOSAvoidROSNamespaceConventionsPrompt"
      mask help: ros:slros:blockmask:SubscriberDescription
      mask init:
      | ros.slros2.internal.block.SubscribeBlockMask.dispatch('maskInitialize', gcb);
      settings: ModelCloseFcn=ros.slros2.internal.bus.Util.clearSLBusesInGlobalScope(gcb);
      mask Help: eval('ros.slros.internal.helpview(''ros2SubscribeBlock'')');
      mask TypeOptions topicSource: ros:slros2:blockmask:TopicSourceFromNetwork | ros:slros2:blockmask:TopicSourceSpecifyOwn
      mask Callback topicSource: ros.slros2.internal.block.SubscribeBlockMask.dispatch('topicSourceSelect', gcb);
      mask Callback topic: ros.slros2.internal.block.SubscribeBlockMask.dispatch('topicEdit', gcb);
      mask Callback messageType: ros.slros2.internal.block.SubscribeBlockMask.dispatch('messageTypeEdit', gcb);
      mask TypeOptions sampleTime: Constant/SampleTime
      mask TypeOptions QOSHistory: SourceBlock/QOSHistory
      mask Callback QOSHistory: ros.slros2.internal.block.QOSSettingsMask.qosHistorySelect(gcb);
      mask TypeOptions QOSDepth: SourceBlock/QOSDepth
      mask TypeOptions QOSReliability: SourceBlock/QOSReliability
      mask TypeOptions QOSDurability: SourceBlock/QOSDurability
      mask TypeOptions QOSDeadline: SourceBlock/QOSDeadline
      mask TypeOptions QOSLifespan: SourceBlock/QOSLifespan
      mask TypeOptions QOSLiveliness: SourceBlock/QOSLiveliness
      mask TypeOptions QOSLeaseDuration: SourceBlock/QOSLeaseDuration
      mask TypeOptions QOSAvoidROSNamespaceConventions: SourceBlock/QOSAvoidROSNamespaceConventions
      mask DialogControl id_netAddrLink Prompt: ros:slros2:blockmask:ConfigNetworkAddrLinkText
      mask DialogControl id_netAddrLink Callback: ros.slros2.internal.block.SubscribeBlockMask.dispatch('configureNetworkAddrDlg', gcb);
      mask DialogControl Container13 Prompt: ros:slros2:blockmask:PubSubMainTab
      mask DialogControl topicSource Prompt: Topic source:
      mask DialogControl topic Prompt: Topic:
      mask DialogControl id_topicSelectBtn Prompt: ros:slros:blockmask:SelectPrompt
      mask DialogControl id_topicSelectBtn Callback: ros.slros2.internal.block.SubscribeBlockMask.dispatch('topicSelect', gcb, 'ros.slros2.internal.dlg.TopicSelector');
      mask DialogControl messageType Prompt: Message type:
      mask DialogControl id_msgTypeSelectBtn Prompt: ros:slros:blockmask:SelectPrompt
      mask DialogControl id_msgTypeSelectBtn Callback: ros.slros2.internal.block.SubscribeBlockMask.dispatch('messageTypeSelect', gcb, 'ros.slros2.internal.dlg.MessageTypeSelector');
      mask DialogControl sampleTime Prompt: Sample time:
      mask DialogControl id_cgContainer Prompt: ros:slros2:blockmask:PubSubQOSTab
      mask DialogControl QOSHistory Prompt: History:
      mask DialogControl QOSDepth Prompt: Depth:
      mask DialogControl QOSReliability Prompt: Reliability:
      mask DialogControl QOSDurability Prompt: Durability:
      mask DialogControl QOSDeadline Prompt: Deadline:
      mask DialogControl QOSLifespan Prompt: Lifespan:
      mask DialogControl QOSLiveliness Prompt: Liveliness:
      mask DialogControl QOSLeaseDuration Prompt: Lease Duration:
      mask DialogControl QOSAvoidROSNamespaceConventions Prompt: Avoid ROS Namespace Conventions
      mask Display:
      | color('black');
      | text(0.83, 0.15, '/apriltag_detector/target_position', 'horizontalAlignment', 'right');
      | port_label('output', 1, 'IsNew');
      | port_label('output', 2, 'Msg');
  Unpack : MATLAB Function  TreatAsAtomicUnit=on
  target_is_new : Outport
  target_data : Outport  Port=2
  target_count : Outport  Port=3
  target_age : Outport  Port=4
  wires:
  Unpack/1(target_data) -> target_data/1
  Unpack/2(target_count) -> target_count/1
  Unpack/3(target_age) -> target_age/1
  Select Data/1 -> Unpack/1(data)  "<data>"
  Clock/1 -> Unpack/3(t)
  Subscribe/2(Out2) -> Select Data/1
  Subscribe/1(Out1) -> target_is_new/1, Unpack/2(is_new)

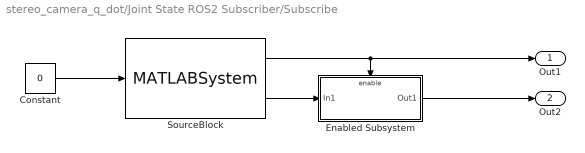
== system stereo_camera_q_dot/Joint State ROS2 Subscriber/Subscribe ==
  Constant : Constant  Value=0  OutDataTypeStr=Bus: SL_Bus_sensor_msgs_JointState  SampleTime=sampleTime  LockScale=on
  Enabled Subsystem : Subsystem  TreatAsAtomicUnit=on
  SourceBlock : MATLABSystem  System=ros.slros2.internal.block.Subscriber  QOSHistory=Keep last  QOSDepth=QOSDepth  QOSReliability=Best effort  QOSDurability=Volatile  QOSDeadline=QOSDeadline  QOSLifespan=QOSLifespan  QOSLiveliness=Automatic  QOSLeaseDuration=QOSLeaseDuration  ROSTopic=/franka/joint_states  ROSMessageType=sensor_msgs/JointState  SLBusName=SL_Bus_sensor_msgs_JointState  ModelName=single_camera_q_dot  BlockId=Sub_single_camera_q_dot_32
      mask Type: ros.slros2.internal.block.Subscriber
  Out1 : Outport  VectorParamsAs1DForOutWhenUnconnected=off
  Out2 : Outport  Port=2  VectorParamsAs1DForOutWhenUnconnected=off
  wires:
  Enabled Subsystem/1(Out1) -> Out2/1
  Constant/1 -> SourceBlock/1
  SourceBlock/2 -> Enabled Subsystem/1(In1)
  SourceBlock/1 -> Out1/1, Enabled Subsystem/Enable

== system stereo_camera_q_dot/Joint Velocity Publisher/Blank Message ==
  Constant : Constant  Value=0  OutDataTypeStr=Bus: SL_Bus_std_msgs_Float64MultiArray  SampleTime=SampleTime  LockScale=on
  Out : Outport  VectorParamsAs1DForOutWhenUnconnected=off  LockScale=on
  wires:
  Constant/1 -> Out/1

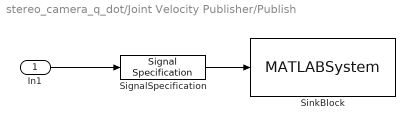
== system stereo_camera_q_dot/Joint Velocity Publisher/Publish ==
  In1 : Inport  LockScale=on
  SignalSpecification : SignalSpecification  OutDataTypeStr=Bus: SL_Bus_std_msgs_Float64MultiArray  BusOutputAsStruct=on
      settings: LockScale=on
  SinkBlock : MATLABSystem  System=ros.slros2.internal.block.Publisher  QOSHistory=Keep last  QOSDepth=QOSDepth  QOSReliability=Reliable  QOSDurability=Volatile  QOSDeadline=QOSDeadline  QOSLifespan=QOSLifespan  QOSLiveliness=Automatic  QOSLeaseDuration=QOSLeaseDuration  ROSTopic=/joint_velocity_example_controller/commands  ROSMessageType=std_msgs/Float64MultiArray  SLBusName=SL_Bus_std_msgs_Float64MultiArray  ModelName=single_camera_q_dot  BlockId=Pub_single_camera_q_dot_351
      mask Type: ros.slros2.internal.block.Publisher
  wires:
  In1/1 -> SignalSpecification/1
  SignalSpecification/1 -> SinkBlock/1

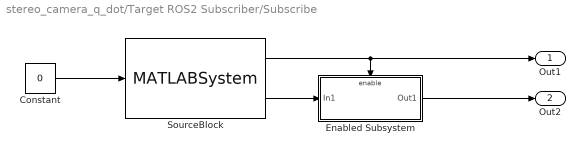
== system stereo_camera_q_dot/Target ROS2 Subscriber/Subscribe ==
  Constant : Constant  Value=0  OutDataTypeStr=Bus: SL_Bus_std_msgs_Float64MultiArray  SampleTime=sampleTime  LockScale=on
  Enabled Subsystem : Subsystem  TreatAsAtomicUnit=on
  SourceBlock : MATLABSystem  System=ros.slros2.internal.block.Subscriber  QOSHistory=Keep last  QOSDepth=QOSDepth  QOSReliability=Best effort  QOSDurability=Volatile  QOSDeadline=QOSDeadline  QOSLifespan=QOSLifespan  QOSLiveliness=Automatic  QOSLeaseDuration=QOSLeaseDuration  ROSTopic=/apriltag_detector/target_position  ROSMessageType=std_msgs/Float64MultiArray  SLBusName=SL_Bus_std_msgs_Float64MultiArray  ModelName=single_camera_q_dot  BlockId=Sub_single_camera_q_dot_22
      mask Type: ros.slros2.internal.block.Subscriber
  Out1 : Outport  VectorParamsAs1DForOutWhenUnconnected=off
  Out2 : Outport  Port=2  VectorParamsAs1DForOutWhenUnconnected=off
  wires:
  Enabled Subsystem/1(Out1) -> Out2/1
  Constant/1 -> SourceBlock/1
  SourceBlock/2 -> Enabled Subsystem/1(In1)
  SourceBlock/1 -> Out1/1, Enabled Subsystem/Enable

== system stereo_camera_q_dot/Joint State ROS2 Subscriber/Subscribe/Enabled Subsystem ==
  note: In Outport bloc, Initial output on outport is 0.
      | This ensures that bus is zeroed out
      | (as the initial condition)
  note: In Enable block, States when enabling = "held".
      | This ensures the "latch" behavior, i.e., this subsystem
      | will output its input when enabled, and its most recent
      | valid input when disabled.
  In1 : Inport
  Enable : EnablePort
  Out1 : Outport  InitialOutput=0  VectorParamsAs1DForOutWhenUnconnected=off
  wires:
  In1/1 -> Out1/1

== system stereo_camera_q_dot/Target ROS2 Subscriber/Subscribe/Enabled Subsystem ==
  note: In Outport bloc, Initial output on outport is 0.
      | This ensures that bus is zeroed out
      | (as the initial condition)
  note: In Enable block, States when enabling = "held".
      | This ensures the "latch" behavior, i.e., this subsystem
      | will output its input when enabled, and its most recent
      | valid input when disabled.
  In1 : Inport
  Enable : EnablePort
  Out1 : Outport  InitialOutput=0  VectorParamsAs1DForOutWhenUnconnected=off
  wires:
  In1/1 -> Out1/1

== matlab function stereo_camera_q_dot/Normalized Image Coordinates/Normalize ==
  data: u input size=1; e output size=[2 1]; v input size=1; z_meas output size=[2 1]; fx parameter size=1; fy parameter size=1; cx parameter size=1; cy parameter size=1; z input
function [e,z_meas] = fcn(u,v, fx, fy, cx, cy,z)
%#codegen
ex=(u-cx)/fx; ey=(v-cy)/fy;
e=[ex;ey]; z_meas=z*e;
end
